simulink model "PAC_experiment"  (R2025a)
settings: Solver=VariableStepAuto  StartTime=0.0  StopTime=200  RelTol=1e-3
undefined symbols (not defined in the file or in its folder): National_Instruments, PCI
libraries: sldrtlib x3, simulink x1
settings Model: Creator=dperera  LastModifiedBy=dperera

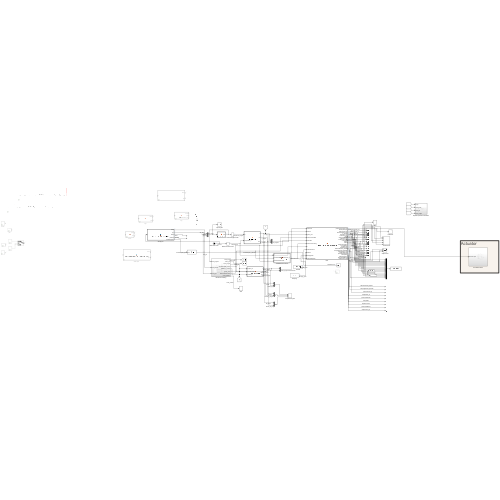
[thumbnail: Simulink's stored preview of the top-level diagram]
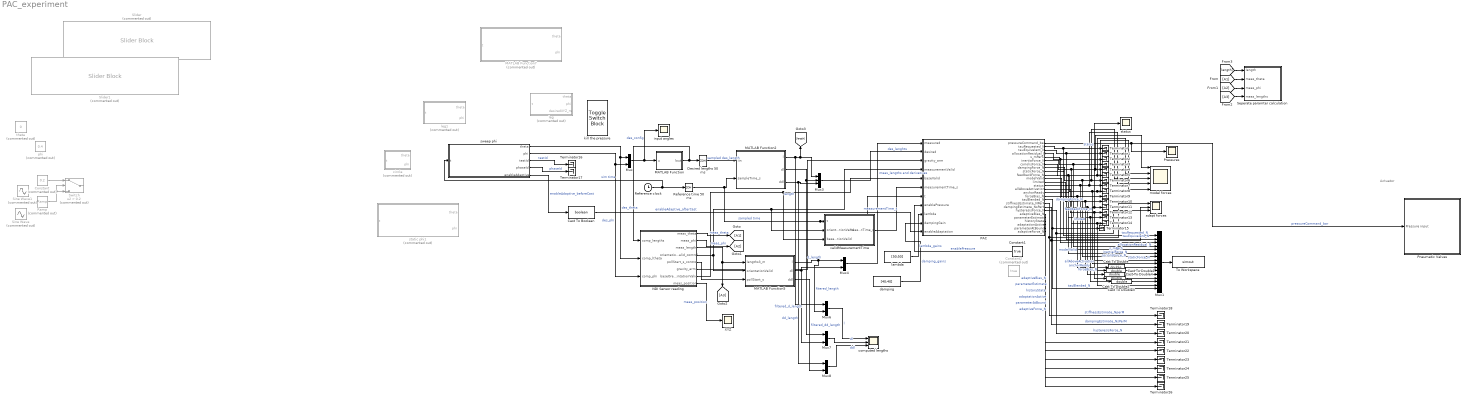
== system PAC_experiment ==
  note: Actuator
  Cast To Boolean : DataTypeConversion  OutDataTypeStr=boolean  SaturateOnIntegerOverflow=off  RndMeth=Floor
  Cast To Double{,1..4} (5 alike) : DataTypeConversion  OutDataTypeStr=double  SaturateOnIntegerOverflow=off  RndMeth=Floor
  Constant : Constant  Commented=on  Value=0.2
  Constant1 : Constant  Value=true  OutDataTypeStr=boolean  SampleTime=0.05
  Constant2 : Constant  Commented=on  Value=true  OutDataTypeStr=boolean
  Desired lengths 50 ms : ZeroOrderHold  SampleTime=0.05
  MATLAB Function : MATLAB Function  TreatAsAtomicUnit=on
  MATLAB Function2 : MATLAB Function  TreatAsAtomicUnit=on
  MATLAB Function5 : MATLAB Function  TreatAsAtomicUnit=on
  MATLAB Function7 : MATLAB Function  Commented=on  TreatAsAtomicUnit=on
  Mux{,4,6..8} (5 alike) : Mux  Inputs=2
  Mux1 : Mux  Inputs=16
  Mux3 : Mux  Inputs=3
  NDI Sensor reading : Subsystem
  PAC : MATLAB Function  TreatAsAtomicUnit=on
  Pneumatic Valves : Subsystem
  Pressures : Scope
      settings: ActiveDisplayYMinimum=-0.31343140031485434  ActiveDisplayYMaximum=2.8208826028336897  DataLoggingVariableName=ScopeData6
  Ramp : simulink/Sources/Ramp  Commented=on  slope=0.2/5  start=1  InitialOutput=0
  Reference clock : Clock
  Reference time 50 ms : ZeroOrderHold  SampleTime=0.05
  Seperate paramter calculation : Subsystem
  Sine Wave : Sin  Commented=on  Amplitude=1.5  Bias=1.5  Frequency=0.2  Phase=3*pi/2  SampleTime=0
  Sine Wave1 : Sin  Commented=on  Amplitude=1.5  Bias=1.5  Frequency=0.2  Phase=3*pi/2  SampleTime=0
  Slider : SliderBlock  Commented=on  ScaleMin=-3.14  ScaleMax=3.14
  Slider1 : SliderBlock  Commented=on  ScaleMax=3.14
  Switch : Switch  Commented=on  Criteria=u2 > Threshold  Threshold=0.2  SaturateOnIntegerOverflow=off  InputSameDT=off
  Terminator{,1..26} (27 alike) : Terminator
  To Workspace : ToWorkspace  VariableName=simout  SaveFormat=Timeseries  SampleTime=-1
  XYZ : Scope
      settings: ActiveDisplayYMinimum=-0.091510816574096682  ActiveDisplayYMaximum=0.32359734916687011  DataLoggingVariableName=ScopeData15
  adapt forces : Scope  NumInputPorts=3
      settings: ActiveDisplayYMinimum=-220.00137487802235  ActiveDisplayYMaximum=1980.0123739022017  DataLoggingVariableName=ScopeData9
  circle : MATLAB Function  Commented=on  TreatAsAtomicUnit=on
  computed lengths : Scope  NumInputPorts=3
      settings: ActiveDisplayYMinimum=-0.010198711471822551  ActiveDisplayYMaximum=0.014062901771668192  DataLoggingVariableName=ScopeData11
  damping : Constant  Value=[40;40]  SampleTime=0.05
  input angles : Scope
      settings: ActiveDisplayYMinimum=-0.19634954084936201  ActiveDisplayYMaximum=1.7671458676442586  DataLoggingVariableName=ScopeData12
  kill the pressure : ToggleSwitchBlock
  lambda : Constant  Value=[50;50]  SampleTime=0.05
  leg : MATLAB Function  Commented=on  TreatAsAtomicUnit=on
  leg1 : MATLAB Function  Commented=on  TreatAsAtomicUnit=on
  model forces : Scope  NumInputPorts=5
      settings: ActiveDisplayYMinimum=-0.19318846896969427  ActiveDisplayYMaximum=0.18409547566465151  DataLoggingVariableName=ScopeData10
  phi : Constant  Commented=on  Value=0.4
  static phi1 : MATLAB Function  Commented=on  TreatAsAtomicUnit=on
  status : Scope
      settings: ActiveDisplayYMinimum=-0.49999999999999989  ActiveDisplayYMaximum=4.5  DataLoggingVariableName=ScopeData8
  sweep phi : MATLAB Function  TreatAsAtomicUnit=on
  theta : Constant  Commented=on  Value=0
  validMeasurementTime : MATLAB Function  TreatAsAtomicUnit=on
  wires:
  Mux/1 -> input angles/1, MATLAB Function/1(u)  "des_config"
  MATLAB Function/1(lout) -> Desired lengths 50 ms/1, NDI Sensor reading/1(comp_lengths)
  NDI Sensor reading/3(meas_length) -> MATLAB Function5/1(lengths3_m), [A3]
  MATLAB Function2/1(l) -> Mux6/1, Mux3/1, [length]  "length"
  MATLAB Function2/2(dl) -> Mux7/1, Mux3/2  "d_length"
  MATLAB Function2/3(ddl) -> Mux8/1, Mux3/3  "dd_length"
  MATLAB Function5/1(l) -> Mux6/2, Mux4/1  "fitered_length"
  MATLAB Function5/2(dl) -> Mux7/2, Mux4/2  "filtered_d_length"
  MATLAB Function5/3(ddl) -> Mux8/2  "filtered_dd_length"
  Desired lengths 50 ms/1 -> MATLAB Function2/1(lIn)  "sampled des_length"
  Reference clock/1 -> sweep phi/1(t), Reference time 50 ms/1  "sim time"
  Reference time 50 ms/1 -> PAC/7(t), validMeasurementTime/1(t), MATLAB Function2/2(sampleTime_s)  "sampled time"
  NDI Sensor reading/4(orientationValid_control) -> MATLAB Function5/2(orientationValid), validMeasurementTime/2(orientationValid), PAC/4(measurementValid)
  NDI Sensor reading/5(pollStart_s_control) -> MATLAB Function5/3(pollStart_s)
  NDI Sensor reading/1(meas_theta) -> [A1]  "meas_theta"
  [A1] -> Seperate paramter calculation/2(meas_theta)
  NDI Sensor reading/2(meas_phi) -> [A2]  "meas_phi"
  [A2] -> Seperate paramter calculation/3(meas_phi)
  [A3] -> Seperate paramter calculation/4(meas_lengths)
  [length] -> Seperate paramter calculation/1(length)
  Mux6/1 -> computed lengths/1  "l"
  Mux7/1 -> computed lengths/2  "dl"
  Mux8/1 -> computed lengths/3  "ddl"
  Ramp/1 -> Switch/2, Switch/3
  Constant/1 -> Switch/1
  sweep phi/2(phi) -> NDI Sensor reading/3(comp_phi), Mux/2  "des_phi"
  sweep phi/1(theta) -> NDI Sensor reading/2(comp_ltheta), Mux/1  "des_theta"
  NDI Sensor reading/8(meas_position) -> XYZ/1  "meas_position"
  PAC/1(pressureCommand_bar) -> Pressures/1, Pneumatic Valves/1(Pressure input)  "pressureCommand_bar"
  Mux4/1 -> PAC/1(measured)  "meas_lengths and derivatives"
  Mux3/1 -> PAC/2(desired)  "des_lenghts"
  NDI Sensor reading/6(gravity_arm) -> PAC/3(gravity_arm)
  NDI Sensor reading/7(baseOreintationValid) -> validMeasurementTime/3(baseOrientationValid), PAC/5(baseValid)
  validMeasurementTime/1(measurementTime_s) -> PAC/6(measurementTime_s)  "measurementTime_s"
  Constant1/1 -> PAC/8(enablePressure)  "enablePressure"
  PAC/2(tauRequested_N) -> Terminator/1, Mux1/1  "tauRequested_N"
  PAC/3(tauEquivalent_N) -> Terminator1/1, Mux1/2  "tauEquivalent_N"
  PAC/4(allocationResidual_N) -> Terminator2/1, Mux1/3  "allocationResidual_N"
  PAC/5(s_mPerS) -> Mux1/4, Terminator3/1  "s_mPerS"
  PAC/6(inertiaForce_N) -> model forces/1, Terminator4/1, Mux1/5  "inertialForce_N"
  PAC/7(coriolisForce_N) -> model forces/2, Terminator5/1, Mux1/6  "coriolisForce_N"
  PAC/8(dampingForce_N) -> Mux1/7, model forces/3, Terminator6/1  "dampingForce_N"
  PAC/9(staticForce_N) -> model forces/4, Terminator7/1, Mux1/8  "staticForce_N"
  PAC/10(feedbackForce_N) -> Mux1/9, model forces/5, Terminator8/1  "feedbackForce_N"
  PAC/11(modelValid) -> Terminator9/1, Cast To Double/1  "modelValid"
  PAC/12(limited) -> Terminator10/1, Cast To Double1/1  "limited"
  PAC/13(status) -> status/1, Terminator11/1, Cast To Double4/1  "status"
  PAC/14(allAboveActivation) -> Cast To Double2/1, Terminator12/1  "allAboveActivation"
  PAC/15(anchorReady) -> Terminator13/1, Cast To Double3/1  "anchorReady"
  PAC/16(forceBias_N) -> Mux1/15, Terminator14/1  "forceBias_N"
  PAC/17(tauBlended_N) -> Terminator15/1, Mux1/16  "tauBlended_N"
  Mux1/1 -> To Workspace/1
  Cast To Double/1 -> Mux1/10
  Cast To Double1/1 -> Mux1/11
  Cast To Double2/1 -> Mux1/13
  Cast To Double3/1 -> Mux1/14
  Cast To Double4/1 -> Mux1/12
  lambda/1 -> PAC/9(lambda)  "lambda_gains"
  damping/1 -> PAC/10(dampingGain)  "damping_gains"
  PAC/18(stiffnessEstimate_NPerM) -> adapt forces/1, Terminator18/1  "stiffnessEstimate_NperM"
  PAC/19(dampingEstimate_NsPerM) -> adapt forces/2, Terminator19/1  "dampingEstimate_NsPerM"
  PAC/20(hysteresisForce_N) -> adapt forces/3, Terminator20/1  "hysteresisForce_N"
  PAC/21(adaptiveBias_N) -> Terminator21/1  "adaptiveBias_N"
  PAC/22(parameterEstimate) -> Terminator22/1  "parameterEstimate"
  PAC/23(historyState) -> Terminator23/1  "historyState"
  PAC/24(adaptationActive) -> Terminator24/1  "adaptationActive"
  PAC/25(parameterAtBound) -> Terminator25/1  "parameterAtBound"
  PAC/26(adaptiveForce_N) -> Terminator26/1  "adaptiveForce_N"
  sweep phi/3(testId) -> Terminator16/1  "testId"
  sweep phi/4(phaseId) -> Terminator17/1  "phaseId"
  sweep phi/5(enableAdaptive) -> Cast To Boolean/1  "enableAdaptive_beforeCast"
  Cast To Boolean/1 -> PAC/11(enableAdaptation)  "enableAdaptive_afterCast"

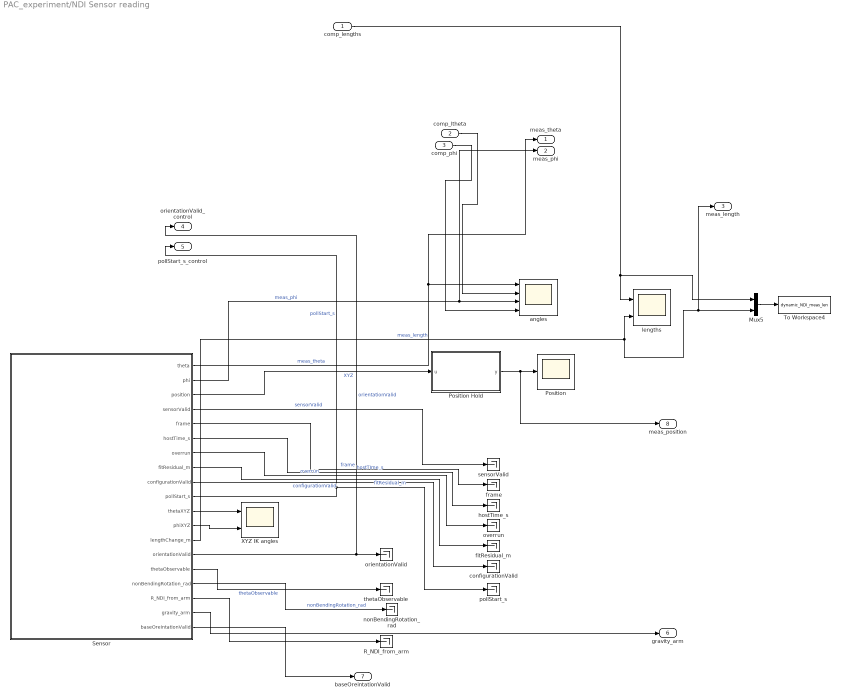
== system PAC_experiment/NDI Sensor reading ==
  comp_lengths : Inport
  comp_ltheta : Inport  Port=2
  comp_phi : Inport  Port=3
  Mux5 : Mux  Inputs=2
  Position : Scope
      settings: ActiveDisplayYMinimum=-0.21656345474719998  ActiveDisplayYMaximum=0.33777835857868188
  Position Hold : MATLAB Function  TreatAsAtomicUnit=on
  R_NDI_from_arm : Terminator
  Sensor : Subsystem
  To Workspace4 : ToWorkspace  VariableName=dynamic_NDI_meas_len  SaveFormat=Timeseries  SampleTime=-1
  XYZ IK angles : Scope  NumInputPorts=2
      settings: DataLoggingVariableName=ScopeData2
  angles : Scope  NumInputPorts=4
      settings: ActiveDisplayYMinimum=-1.199121055664828  ActiveDisplayYMaximum=1.8446149853511815
  configurationValid : Terminator
  fitResidual_m : Terminator
  frame : Terminator
  hostTime_s : Terminator
  lengths : Scope  NumInputPorts=2
      settings: ActiveDisplayYMinimum=-0.0017146774565175815  ActiveDisplayYMaximum=0.0020057370608089205  DataLoggingVariableName=ScopeData3
  nonBendingRotation_rad : Terminator
  orientationValid : Terminator
  overrun : Terminator
  pollStart_s : Terminator
  sensorValid : Terminator
  thetaObservable : Terminator
  meas_theta : Outport
  meas_phi : Outport  Port=2
  meas_length : Outport  Port=3
  orientationValid_control : Outport  Port=4
  pollStart_s_control : Outport  Port=5
  gravity_arm : Outport  Port=6
  baseOreintationValid : Outport  Port=7
  meas_position : Outport  Port=8
  wires:
  Sensor/13(lengthChange_m) -> lengths/2, meas_length/1, Mux5/2  "meas_length"
  comp_lengths/1 -> lengths/1, Mux5/1
  Sensor/10(pollStart_s) -> pollStart_s_control/1, pollStart_s/1  "pollStart_s"
  Sensor/2(phi) -> angles/3, meas_phi/1  "meas_phi"
  Sensor/3(position) -> Position Hold/1(u)  "XYZ"
  Sensor/1(theta) -> meas_theta/1, angles/1  "meas_theta"
  Sensor/6(hostTime_s) -> hostTime_s/1  "hostTIme_s"
  Sensor/9(configurationValid) -> configurationValid/1  "configurationValid"
  Sensor/4(sensorValid) -> sensorValid/1  "sensorValid"
  Sensor/7(overrun) -> overrun/1  "overrun"
  Sensor/5(frame) -> frame/1  "frame"
  comp_ltheta/1 -> angles/2
  Sensor/8(fitResidual_m) -> fitResidual_m/1  "fitResidual_m"
  Sensor/12(phiXYZ) -> XYZ IK angles/2
  Sensor/11(thetaXYZ) -> XYZ IK angles/1
  Position Hold/1(y) -> meas_position/1, Position/1
  Mux5/1 -> To Workspace4/1
  Sensor/14(orientationValid) -> orientationValid_control/1, orientationValid/1  "orientationValid"
  Sensor/16(nonBendingRotation_rad) -> nonBendingRotation_rad/1  "nonBendingRotation_rad"
  Sensor/15(thetaObservable) -> thetaObservable/1  "thetaObservable"
  comp_phi/1 -> angles/4
  Sensor/19(baseOreintationValid) -> baseOreintationValid/1
  Sensor/17(R_NDI_from_arm) -> R_NDI_from_arm/1
  Sensor/18(gravity_arm) -> gravity_arm/1

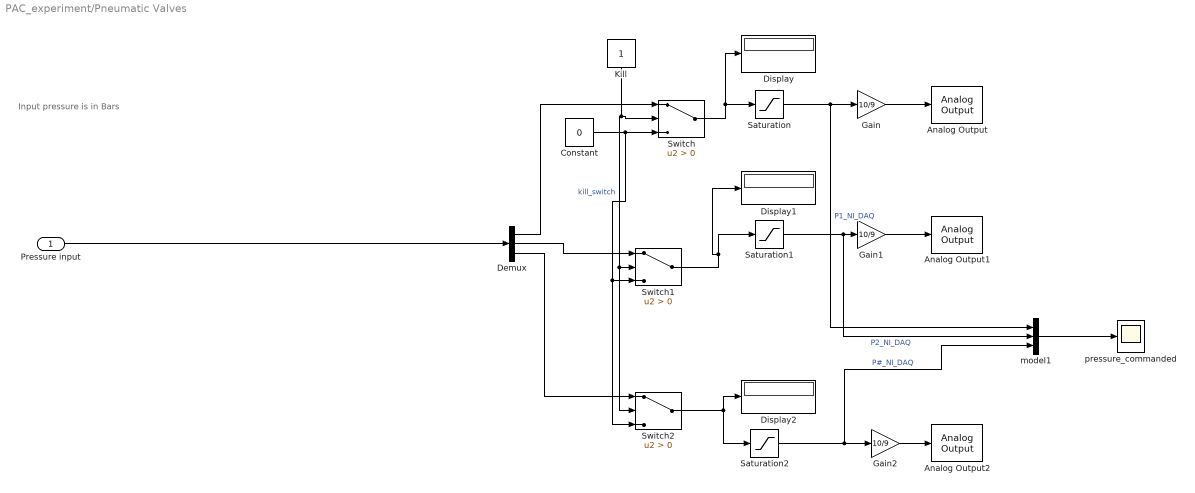
== system PAC_experiment/Pneumatic Valves ==
  note: Input pressure is in Bars
  Pressure input : Inport
  Analog Output : sldrtlib/Analog Output  SampleTime=1/100  MaxMissedTicks=inf  ShowMissedTicks=off  YieldWhenWaiting=off  DrvName=National_Instruments/PCI-6703  DrvAddress=4294967295  DrvOptions=0  Channels=1  RangeMode=1  VoltRange=1  InitialValue=0  FinalValue=0
      settings: AttributesFormatString=National Instruments\nPCI-6703 [auto]
  Analog Output1 : sldrtlib/Analog Output  SampleTime=1/100  MaxMissedTicks=inf  ShowMissedTicks=off  YieldWhenWaiting=off  DrvName=National_Instruments/PCI-6703  DrvAddress=4294967295  DrvOptions=0  Channels=2  RangeMode=1  VoltRange=1  InitialValue=0  FinalValue=0
      settings: AttributesFormatString=National Instruments\nPCI-6703 [auto]
  Analog Output2 : sldrtlib/Analog Output  SampleTime=1/100  MaxMissedTicks=inf  ShowMissedTicks=off  YieldWhenWaiting=off  DrvName=National_Instruments/PCI-6703  DrvAddress=4294967295  DrvOptions=0  Channels=3  RangeMode=1  VoltRange=1  InitialValue=0  FinalValue=0
      settings: AttributesFormatString=National Instruments\nPCI-6703 [auto]
  Constant : Constant  Value=0
  Demux : Demux  Outputs=3
  Display : Display
  Display1 : Display
  Display2 : Display
  Gain : Gain  Gain=10/9
  Gain1 : Gain  Gain=10/9
  Gain2 : Gain  Gain=10/9
  Kill : Constant
  Saturation : Saturate  UpperLimit=3  LowerLimit=0
  Saturation1 : Saturate  UpperLimit=3  LowerLimit=0
  Saturation2 : Saturate  UpperLimit=3  LowerLimit=0
  Switch : Switch  Criteria=u2 > Threshold  SaturateOnIntegerOverflow=off  InputSameDT=off
  Switch1 : Switch  Criteria=u2 > Threshold  SaturateOnIntegerOverflow=off  InputSameDT=off
  Switch2 : Switch  Criteria=u2 > Threshold  SaturateOnIntegerOverflow=off  InputSameDT=off
  model1 : Mux  Inputs=3
  pressure_commanded : Scope
      settings: ActiveDisplayYMinimum=-0.37499999999999989  ActiveDisplayYMaximum=3.375  DataLoggingVariableName=ScopeData7
  wires:
  Constant/1 -> Switch2/3, Switch1/3, Switch/3
  Kill/1 -> Switch2/2, Switch1/2, Switch/2  "kill_switch"
  Switch/1 -> Display/1, Saturation/1
  Gain/1 -> Analog Output/1
  Saturation/1 -> model1/1, Gain/1  "P1_NI_DAQ"
  Demux/3 -> Switch2/1
  Gain1/1 -> Analog Output1/1
  Gain2/1 -> Analog Output2/1
  Saturation2/1 -> model1/3, Gain2/1  "P#_NI_DAQ"
  Switch2/1 -> Saturation2/1, Display2/1
  Demux/2 -> Switch1/1
  Switch1/1 -> Saturation1/1, Display1/1
  model1/1 -> pressure_commanded/1
  Saturation1/1 -> model1/2, Gain1/1  "P2_NI_DAQ"
  Demux/1 -> Switch/1
  Pressure input/1 -> Demux/1

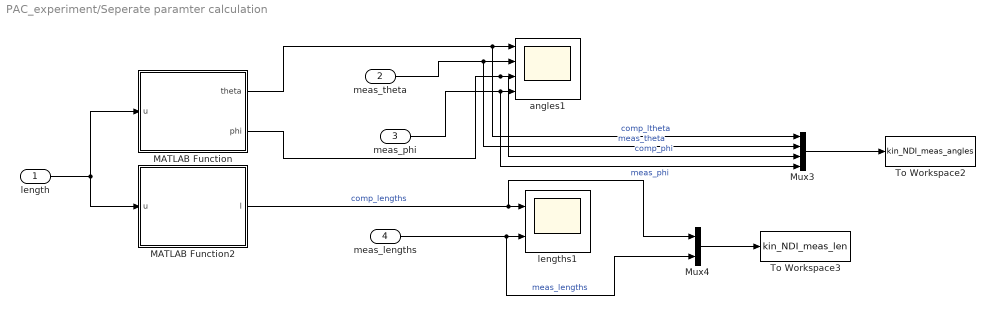
== system PAC_experiment/Seperate paramter calculation ==
  length : Inport
  meas_theta : Inport  Port=2
  meas_phi : Inport  Port=3
  meas_lengths : Inport  Port=4
  MATLAB Function : MATLAB Function  TreatAsAtomicUnit=on
  MATLAB Function2 : MATLAB Function  TreatAsAtomicUnit=on
  Mux3 : Mux
  Mux4 : Mux  Inputs=2
  To Workspace2 : ToWorkspace  VariableName=kin_NDI_meas_angles  SaveFormat=Timeseries  SampleTime=-1
  To Workspace3 : ToWorkspace  VariableName=kin_NDI_meas_len  SaveFormat=Timeseries  SampleTime=-1
  angles1 : Scope  NumInputPorts=4
      settings: ActiveDisplayYMinimum=-3.9269137322662839  ActiveDisplayYMaximum=3.9265599408279468  DataLoggingVariableName=ScopeData4
  lengths1 : Scope  NumInputPorts=2
      settings: ActiveDisplayYMinimum=-0.02243223759551808  ActiveDisplayYMaximum=0.037530111947788623  DataLoggingVariableName=ScopeData5
  wires:
  meas_lengths/1 -> Mux4/2, lengths1/2  "meas_lengths"
  meas_theta/1 -> Mux3/2, angles1/2  "meas_theta"
  MATLAB Function/2(phi) -> Mux3/3, angles1/3  "comp_phi"
  Mux3/1 -> To Workspace2/1
  meas_phi/1 -> Mux3/4, angles1/4  "meas_phi"
  MATLAB Function/1(theta) -> Mux3/1, angles1/1  "comp_ltheta"
  Mux4/1 -> To Workspace3/1
  MATLAB Function2/1(l) -> Mux4/1, lengths1/1  "comp_lengths"
  length/1 -> MATLAB Function2/1(u), MATLAB Function/1(u)

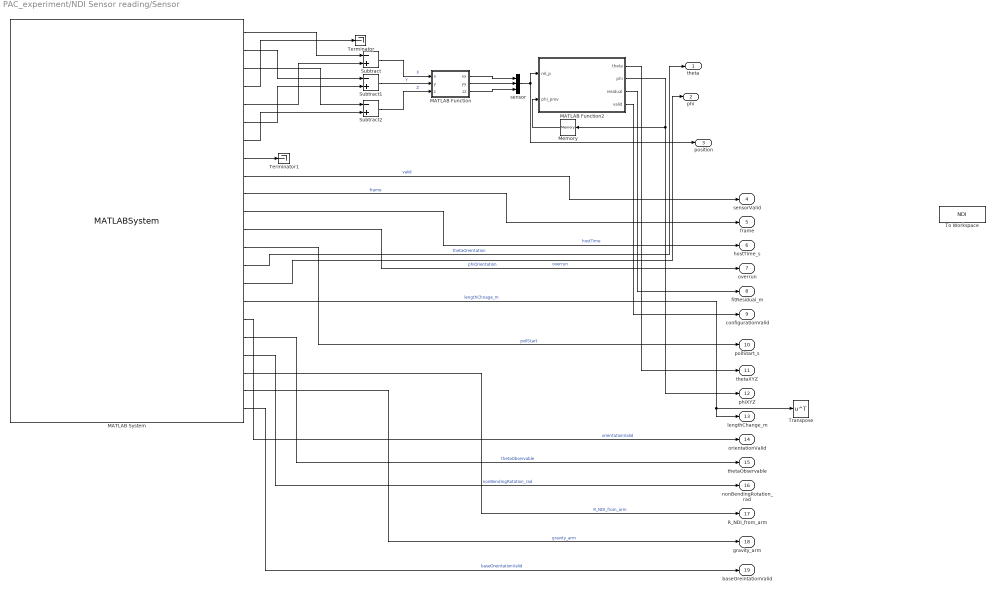
== system PAC_experiment/NDI Sensor reading/Sensor ==
  MATLAB Function : MATLAB Function  TreatAsAtomicUnit=on
  MATLAB Function2 : MATLAB Function  TreatAsAtomicUnit=on
  MATLAB System : MATLABSystem  System=AuroraReader_s2_BaseRotation  Port=COM12  BaudRate=921600  SamplePeriod=0.05  BaseSensorId=0A  TipSensorId=0B  CalibrationFile=C:\Users\dperera\OneDrive - Texas A&M University\Lab\Research\fDyn_ExpCom\hyDyn_Ctrl\ndi_orientation_recordings\calibration_20260930_190505_898.mat  PreflightSeconds=5  ActuatorRadius=0.013  ReferenceGravity_arm=[ 0; 0; -9.81 ]  SimulateUsing=Interpreted execution
      mask Type: AuroraReader_s2_BaseRotation
  Memory : Memory  InitialCondition=0.0001
  Subtract : Sum  Inputs=-+
  Subtract1 : Sum  Inputs=-+
  Subtract2 : Sum  Inputs=-+
  Terminator : Terminator
  Terminator1 : Terminator
  To Workspace : ToWorkspace  VariableName=NDI  SaveFormat=Timeseries  SampleTime=-1
  Transpose : Math  Operator=transpose
  sensor : Mux  Inputs=3
  theta : Outport
  phi : Outport  Port=2
  position : Outport  Port=3
  sensorValid : Outport  Port=4
  frame : Outport  Port=5
  hostTime_s : Outport  Port=6
  overrun : Outport  Port=7
  fitResidual_m : Outport  Port=8
  configurationValid : Outport  Port=9
  pollStart_s : Outport  Port=10
  thetaXYZ : Outport  Port=11
  phiXYZ : Outport  Port=12
  lengthChange_m : Outport  Port=13
  orientationValid : Outport  Port=14
  thetaObservable : Outport  Port=15
  nonBendingRotation_rad : Outport  Port=16
  R_NDI_from_arm : Outport  Port=17
  gravity_arm : Outport  Port=18
  baseOreintationValid : Outport  Port=19
  wires:
  MATLAB System/2 -> Subtract1/1
  MATLAB Function/3(zz) -> sensor/3
  Subtract1/1 -> MATLAB Function/2(y)  "Y"
  Subtract2/1 -> MATLAB Function/3(z)  "Z"
  MATLAB System/5 -> Subtract/2
  sensor/1 -> position/1, MATLAB Function2/1(rel_p)
  MATLAB System/8 -> Terminator1/1
  MATLAB Function/1(xx) -> sensor/1
  Subtract/1 -> MATLAB Function/1(x)  "X"
  MATLAB Function/2(yy) -> sensor/2
  MATLAB System/1 -> Subtract/1
  MATLAB Function2/2(phi) -> Memory/1, phiXYZ/1
  MATLAB System/7 -> Subtract2/2
  MATLAB System/4 -> Terminator/1
  MATLAB System/3 -> Subtract2/1
  MATLAB System/6 -> Subtract1/2
  Memory/1 -> MATLAB Function2/2(phi_prev)
  MATLAB System/9 -> sensorValid/1  "valid"
  MATLAB System/11 -> hostTime_s/1  "hostTime"
  MATLAB System/12 -> overrun/1  "overrun"
  MATLAB Function2/3(residual) -> fitResidual_m/1
  MATLAB Function2/4(valid) -> configurationValid/1
  MATLAB System/13 -> pollStart_s/1  "pollStart"
  MATLAB System/14 -> theta/1  "thetaOrientation"
  MATLAB System/15 -> phi/1  "phiOrientation"
  MATLAB Function2/1(theta) -> thetaXYZ/1
  MATLAB System/16 -> lengthChange_m/1, Transpose/1  "lengthChnage_m"
  MATLAB System/17 -> orientationValid/1  "orientationValid"
  MATLAB System/18 -> thetaObservable/1  "thetaObservable"
  MATLAB System/19 -> nonBendingRotation_rad/1  "nonBendingRotation_rad"
  MATLAB System/10 -> frame/1  "frame"
  MATLAB System/20 -> R_NDI_from_arm/1  "R_NDI_from_arm"
  MATLAB System/21 -> gravity_arm/1  "gravity_arm"
  MATLAB System/22 -> baseOreintationValid/1  "baseOreintationValid"

== matlab function PAC_experiment/Seperate paramter calculation/MATLAB Function ==
  data: u input; theta output; phi output
function [theta, phi] = length2config(u)
%#codegen
% This file convert the length changes into theta/phi
%
% Inputs:
%   u       : length change[2x1] (m)
%             [l2; l3]
%
% Outputs:
%   theta   : bending direction [constant] (rad)
%   phi     : bending amount [constant] (rad)

l = [0.0; u(1); u(2)];
r  = 0.013;

c = [atan2(l(3) - l(2), sqrt(0.3e1) * (l(2) + l(3)));
    0.2e1 / 0.3e1 / r * sqrt((3 * l(2) ^ 2 + 3 * l(3) * l(2) + 3 * l(3) ^ 2))];

theta = c(1);
phi = c(2);

end

== matlab function PAC_experiment/Seperate paramter calculation/MATLAB Function2 ==
  data: u input; l output
function l = lengthVector(u)
%#codegen
% This file create the length vector
%
% Inputs:
%   u       : length change[2x1] (m)
%             [l2; l3]
%
% Outputs:
%   l   : bending direction [3x1] (m)

l = [-(u(1) + u(2)); u(1); u(2)];

end

== matlab function PAC_experiment/NDI Sensor reading/Position Hold ==
  data: u input; y output
function y = fcn(u)
persistent lastPosition
if isempty(lastPosition), lastPosition=nan(3,1); end
if all(isfinite(u)), lastPosition=u; end
y=lastPosition;
end

== matlab function PAC_experiment/NDI Sensor reading/Sensor/MATLAB Function ==
  data: x input; xx output; y input; z input; yy output; zz output
function [xx,yy,zz] = rotateX90(x,y,z)

    R = [1 0 0;
         0 0 1;
         0 -1 0];

    p = R*[x;y;z]*0.001;

    xx=p(1);
    yy=p(2);
    zz=p(3);

    
end

== matlab function PAC_experiment/NDI Sensor reading/Sensor/MATLAB Function2 ==
  data: rel_p input; theta output; phi output; phi_prev input; residual output; valid output
function [theta,phi,residual,valid] = xyz2ThetaPhi(rel_p,phi_prev)
persistent lastPhi lastTheta lastOutputTheta lastOutputPhi lastResidual
if isempty(lastPhi)
    lastPhi=0.0001; lastTheta=0;
    lastOutputTheta=NaN; lastOutputPhi=NaN; lastResidual=NaN;
end
% Keep the external memory for compatibility; never use its NaN.
if isfinite(phi_prev), lastPhi=phi_prev; end
[theta,phi,residual,valid]=ndiSupportFnc.configuration(rel_p,lastPhi,lastTheta);
if valid
    lastPhi=phi; lastTheta=theta;
    lastOutputTheta=theta; lastOutputPhi=phi; lastResidual=residual;
else
    % Scope outputs hold, but configurationValid remains false.
    theta=lastOutputTheta; phi=lastOutputPhi; residual=lastResidual;
end
end

== matlab function PAC_experiment/MATLAB Function ==
  data: u input; lout output
function lout = config2length(u)
%#codegen
% Convert configuration variables to length changes
% Input (u):
%   u       : theta and phi [2x1] (rad)
%               theta angle (rad) [constant]
%               phi angle (rad) [constant]
%   r       : radial offset (m) [constant]
% 
% Output:
%   lout    : lenght changes (m) [s,1]


theta = u(1);
phi = u(2);
r = 0.013;

l = [-r * cos(theta) * phi;
    (0.5e0 * r * cos(theta) - sqrt(0.3e1) * r * sin(theta) / 0.2e1) * phi;
    (0.5e0 * r * cos(theta) + sqrt(0.3e1) * r * sin(theta) / 0.2e1) * phi];

lout = [l(2); l(3)];

end

== matlab function PAC_experiment/MATLAB Function2 ==
  data: lIn input; l output; dl output; ddl output; sampleTime_s input
function [l, dl, ddl] = lengthDerivatives(lIn, sampleTime_s)
%#codegen
% Desired reduced lengths [l2;l3] in m; derivatives in m/s and m/s^2.
% sampleTime_s is a 0.05 s zero-order-held Clock signal.
persistent lastL lastT velocity acceleration
if isempty(lastT)
    lastL = zeros(2,1);
    lastT = -1;
    velocity = zeros(2,1);
    acceleration = zeros(2,1);
end
l = lastL;
dl = velocity;
ddl = acceleration;
if ~all(isfinite(lIn)) || ~isfinite(sampleTime_s)
    return;
end
q = [lIn(1); lIn(2)];
if lastT < 0
    lastL = q;
    lastT = sampleTime_s;
    l = q;
    return;
end
dt = sampleTime_s - lastT;
if dt > 1e-6
    rawVelocity = (q-lastL)/dt;
    oldVelocity = velocity;
    alphaV = dt/(0.10+dt);
    velocity = velocity + alphaV*(rawVelocity-velocity);
    rawAcceleration = (velocity-oldVelocity)/dt;
    alphaA = dt/(0.15+dt);
    acceleration = acceleration + alphaA*(rawAcceleration-acceleration);
    lastL = q;
    lastT = sampleTime_s;
end
l = lastL;
dl = velocity;
ddl = acceleration;
end

== matlab function PAC_experiment/validMeasurementTime ==
  data: t input; measurementTime_s output; orientationValid input; baseOrientationValid input
function measurementTime_s = validMeasurementTime( ...
    t, orientationValid, baseOrientationValid)
%#codegen

persistent lastValidTime
if isempty(lastValidTime)
    lastValidTime = -1.0;
end

if orientationValid && baseOrientationValid && isfinite(t)
    lastValidTime = t;
end

measurementTime_s = lastValidTime;
end

== matlab function PAC_experiment/sweep phi ==
  data: t input; theta output; phi output; testId output; phaseId output; enableAdaptive output
function [theta,phi,testId,phaseId, enableAdaptive] = pacStaticSweepReferenceBlock(t)
%#codegen
% Paste into reference MATLAB Function block. All settings are internal.
% 10 trials: three amplitudes in three directions, then repeat theta=0/.2.
% Stop Time 535 s. Start only if controller status=3 before 25 s.
% Learn normally, then freeze before the 0.8-rad unloading at 110 s.
adaptationFreezeTime_s = 105.0;
enableAdaptive = isfinite(t) && t >= 0.0 && ...
                 t < adaptationFreezeTime_s;
start_s=25.0;
rise_s=5.0; hold_s=30.0; fall_s=5.0; zeroHold_s=10.0;
thetaList=[0 0 0 pi/2 pi/2 pi/2 pi pi pi 0];
phiList=[.5 .8 1.0 .5 .8 1.0 .5 .8 1.0 .5];
theta=0.0;phi=0.0;testId=0.0;phaseId=0.0;
if ~isfinite(t) || t<start_s, return; end
trial_s=rise_s+hold_s+fall_s+zeroHold_s;
idx=floor((t-start_s)/trial_s)+1;
if idx>numel(phiList),return;end
testId=double(idx);theta=thetaList(idx);
local=t-start_s-(idx-1)*trial_s;
if local<rise_s
    phaseId=1.0;u=local/rise_s;phi=phiList(idx)*u*u*(3-2*u);
elseif local<rise_s+hold_s
    phaseId=2.0;phi=phiList(idx);
elseif local<rise_s+hold_s+fall_s
    phaseId=3.0;u=(local-rise_s-hold_s)/fall_s;
    phi=phiList(idx)*(1-u*u*(3-2*u));
else
    phaseId=4.0;
end
end

== matlab function PAC_experiment/MATLAB Function5 ==
  data: lengths3_m input; l output; dl output; ddl output; orientationValid input; pollStart_s input
function [l, dl, ddl] = filteredDerivatives(lengths3_m, orientationValid, pollStart_s)
%#codegen
% NDI lengths are [l1;l2;l3]; model coordinates are [l2;l3].
% Invalid or repeated BX frames do not update the derivative states.
persistent lastL lastT velocity acceleration
if isempty(lastT)
    lastL = nan(2,1);
    lastT = -1;
    velocity = zeros(2,1);
    acceleration = zeros(2,1);
end
l = lastL;
dl = velocity;
ddl = acceleration;
if ~orientationValid || ~all(isfinite(lengths3_m)) || ~isfinite(pollStart_s)
    return;
end
q = [lengths3_m(2); lengths3_m(3)];
if lastT < 0
    lastL = q;
    lastT = pollStart_s;
    l = q;
    return;
end
dt = pollStart_s-lastT;
if dt > 1e-6
    rawVelocity = (q-lastL)/dt;
    oldVelocity = velocity;
    alphaV = dt/(0.20+dt);
    velocity = velocity + alphaV*(rawVelocity-velocity);
    rawAcceleration = (velocity-oldVelocity)/dt;
    alphaA = dt/(0.30+dt);
    acceleration = acceleration + alphaA*(rawAcceleration-acceleration);
    lastL = q;
    lastT = pollStart_s;
end
l = lastL;
dl = velocity;
ddl = acceleration;
end

== matlab function PAC_experiment/static phi1 ==
  data: t input; theta output; phi output
function [theta, phi] = commonPressureFeedbackReferenceBlock(t)
%#codegen
% Fixed-direction ramp-and-hold test.
% Suggested simulation Stop Time: 70 s.

des_phi = 0.2;       % rad
des_theta = 0.0;     % rad
startTime_s = 25.0;  % Allow trim and feedback blend to finish
riseTime_s = 5.0;
holdTime_s = 30.0;
fallTime_s = 5.0;

theta = des_theta;
phi = 0.0;

if ~isfinite(t) || t < 0.0
    return;
end

holdStart_s = startTime_s + riseTime_s;
fallStart_s = holdStart_s + holdTime_s;
endTime_s = fallStart_s + fallTime_s;

if t < startTime_s
    return;
elseif t < holdStart_s
    u = (t - startTime_s)/riseTime_s;
    phi = des_phi*u*u*(3.0 - 2.0*u);
elseif t < fallStart_s
    phi = des_phi;
elseif t < endTime_s
    u = (t - fallStart_s)/fallTime_s;
    phi = des_phi*(1.0 - u*u*(3.0 - 2.0*u));
end
end

== matlab function PAC_experiment/MATLAB Function7 ==
  data: t input; theta output; phi output
function [theta, phi] = commonPressureFeedbackReferenceBlock(t)
%#codegen
% Paste into the existing thetaCircle MATLAB Function block in a COPY of
% the feedback-linearization model. Connect theta and phi to the desired
% angle Mux and NDI comparison inputs; bypass the old circle/ramp sources.
% Stop Time: 240 s. Both reference steps are only 0.01 rad.

theta = 0.0;
phi = 0.0;
if ~isfinite(t) || t < 0.0
    return;
end

if t >= 90.0 && t < 130.0
    theta = 0.0; % U-direction bend.
    if t < 95.0
        u = (t-90.0)/5.0;
        phi = 0.01*u*u*(3.0-2.0*u);
    elseif t < 125.0
        phi = 0.01;
    else
        u = (t-125.0)/5.0;
        phi = 0.01*(1.0-u*u*(3.0-2.0*u));
    end
elseif t >= 160.0 && t < 200.0
    theta = pi/2; % V-direction bend.
    if t < 165.0
        u = (t-160.0)/5.0;
        phi = 0.01*u*u*(3.0-2.0*u);
    elseif t < 195.0
        phi = 0.01;
    else
        u = (t-195.0)/5.0;
        phi = 0.01*(1.0-u*u*(3.0-2.0*u));
    end
end
end

== matlab function PAC_experiment/leg ==
  data: t input; theta output; phi output; desiredXYZ_m output
function [theta, phi, desiredXYZ_m] = square(t)
%#codegen
% One 10 cm x 10 cm square in arm-frame X-Y.
% Z follows the fixed-length, constant-curvature geometry.

side_m = 0.10;
h = side_m/2;

rotationTime_s = 10.0;
trimTime_s = 5.0;
approachTime_s = 10.0;
cornerHold_s = 5.0;
sideTime_s = 5.0;      % time for each 10 cm side
numSquares = 10;         % increase after the first test
returnTime_s = 10.0;

% Base-sensor offset, module length, tip-sensor offset.
Lbase = 0.055;
Lmodule = 0.17411;
Ltip = 0.05;

approachStart_s = rotationTime_s + trimTime_s;
approachEnd_s = approachStart_s + approachTime_s;
squareStart_s = approachEnd_s + cornerHold_s;
squareEnd_s = squareStart_s + 4*numSquares*sideTime_s;
returnEnd_s = squareEnd_s + returnTime_s;

theta = 0.0;
phi = 0.0;
desiredXYZ_m = [0.0; 0.0; Lbase + Lmodule + Ltip];

if ~isfinite(t) || t < approachStart_s
    return;
end

x = 0.0;
y = 0.0;

if t < approachEnd_s
    % Move from straight to the first corner (+h,+h).
    u = (t - approachStart_s)/approachTime_s;
    s = smooth5(u);
    x = h*s;
    y = h*s;
    theta = pi/4;

elseif t < squareStart_s
    % Settle at the first corner.
    x = h;
    y = h;
    theta = pi/4;

elseif t < squareEnd_s
    elapsed = t - squareStart_s;
    lap = floor(elapsed/(4*sideTime_s));
    withinLap = elapsed - lap*(4*sideTime_s);
    side = floor(withinLap/sideTime_s);  % 0, 1, 2, or 3
    u = (withinLap - side*sideTime_s)/sideTime_s;
    s = smooth5(u);

    if side == 0
        x = h - 2*h*s;  y = h;           % (+,+) to (-,+)
    elseif side == 1
        x = -h;         y = h - 2*h*s;   % (-,+) to (-,-)
    elseif side == 2
        x = -h + 2*h*s; y = -h;          % (-,-) to (+,-)
    else
        x = h;          y = -h + 2*h*s;  % (+,-) to (+,+)
    end

    % Keep theta continuous across +/-pi and across laps.
    theta = atan2(y,x);
    if side == 1 && theta < 0.0
        theta = theta + 2*pi;
    elseif side >= 2
        theta = theta + 2*pi;
    end
    theta = theta + 2*pi*lap;

elseif t < returnEnd_s
    % Return from the first corner to straight.
    u = (t - squareEnd_s)/returnTime_s;
    s = smooth5(u);
    x = h*(1.0 - s);
    y = h*(1.0 - s);
    theta = pi/4 + 2*pi*numSquares;

else
    % Remain straight without resetting the unwrapped theta.
    theta = pi/4 + 2*pi*numSquares;
    return;
end

[phi, z] = task2ConfigOnSurface(hypot(x,y), Lbase, Lmodule, Ltip);
desiredXYZ_m = [x; y; z];
end

function s = smooth5(u)
% Zero velocity and acceleration at both ends of each side.
u = min(max(u,0.0),1.0);
s = u*u*u*(10.0 + u*(-15.0 + 6.0*u));
end

function [phi,z] = task2ConfigOnSurface(rho,Lbase,Lmodule,Ltip)
% Invert the same constant-curvature radial geometry as task2config.
% Z is free and is computed from the resulting bend angle.
if rho <= 1e-10
    phi = 0.0;
    z = Lbase + Lmodule + Ltip;
    return;
end

low = 0.0;
high = 1.5;  % rad; comfortably covers this 10 cm square

for k = 1:28
    mid = 0.5*(low + high);
    rhoModel = Lmodule*2.0*sin(mid/2.0)^2/mid ...
             + Ltip*sin(mid);
    if rhoModel < rho
        low = mid;
    else
        high = mid;
    end
end

phi = 0.5*(low + high);
z = Lbase + Lmodule*sin(phi)/phi + Ltip*cos(phi);
end

== matlab function PAC_experiment/circle ==
  data: t input; theta output; phi output
function [theta, phi] = thetaCircle(t)
%#codegen

% Change these values before a run
des_phi = 1.0;             % rad
circle_time_s = 10.0;      % seconds per circle
num_circles = 1;
rotationTime_s = 10.0;     % time available to rotate the base
trimTime_s = 5.0;         % stationary pressure-trim hold
feedbackBlendTime_s = 5.0;
phiRiseTime_s = 5.0;
phiFallTime_s = 5.0;

theta = 0.0;
phi = 0.0;
if ~isfinite(t) || t < 0.0
    return;
end

phiRiseStart_s = rotationTime_s + trimTime_s + feedbackBlendTime_s;
circleStart_s = phiRiseStart_s + phiRiseTime_s;
circleEnd_s = circleStart_s + num_circles*circle_time_s;
phiEnd_s = circleEnd_s + phiFallTime_s;

if t < phiRiseStart_s
    return;
elseif t < circleStart_s
    u = (t - phiRiseStart_s)/phiRiseTime_s;
    phi = des_phi*u*u*(3.0 - 2.0*u);
elseif t < circleEnd_s
    progress = (t - circleStart_s)/circle_time_s;
    lap = floor(progress);
    u = progress - lap;
    theta = 2*pi*(lap + u*u*(3.0 - 2.0*u));
    phi = des_phi;
elseif t < phiEnd_s
    u = (t - circleEnd_s)/phiFallTime_s;
    theta = 2*pi*num_circles;
    phi = des_phi*(1.0 - u*u*(3.0 - 2.0*u));
end
end

== matlab function PAC_experiment/leg1 ==
  data: t input; theta output; phi output
function [theta, phi] = leg(t)
%#codegen

rotationTime_s = 10.0;
trimTime_s = 5.0;
trajectoryStart_s = rotationTime_s + trimTime_s;

% Loaded when the MATLAB Function block compiles.
data = coder.load('Quadruped_leg/Natha_quad_leg_1.mat', ...
                  't', 'leg1_config');
time = data.t;
angles = data.leg1_config;  % row 1: theta; row 2: phi, radians

theta = 0.0;
phi = 0.0;

if ~isfinite(t) || t < trajectoryStart_s
    return;
end

trajectoryTime_s = 0.2 * (t - trajectoryStart_s);

% Hold the final recorded pose after the 40-second trajectory.
if trajectoryTime_s >= time(end)
    theta = angles(1,end);
    phi = angles(2,end);
    return;
end

% Find the two recorded samples surrounding the current time.
lo = 1;
hi = numel(time);
while hi - lo > 1
    mid = floor((lo + hi)/2);
    if trajectoryTime_s < time(mid)
        hi = mid;
    else
        lo = mid;
    end
end

% Linear interpolation between samples.
weight = (trajectoryTime_s - time(lo))/(time(hi) - time(lo));
theta = angles(1,lo) + weight*(angles(1,hi) - angles(1,lo));
phi   = angles(2,lo) + weight*(angles(2,hi) - angles(2,lo));
end

== matlab function PAC_experiment/PAC ==
  settings: sampleTime=0.05
  data: measured input; desired input; gravity_arm input; measurementValid input; baseValid input; measurementTime_s input; t input; pressureCommand_bar output double; tauRequested_N output double; tauEquivalent_N output double; allocationResidual_N output; s_mPerS output; inertiaForce_N output; coriolisForce_N output; dampingForce_N output; staticForce_N output; feedbackForce_N output; modelValid output boolean; limited output boolean; enablePressure input; status output uint8 size=1; allAboveActivation output boolean; anchorReady output boolean; forceBias_N output; tauBlended_N output; lambda input; dampingGain input; enableAdaptation input; stiffnessEstimate_NPerM output; dampingEstimate_NsPerM output; hysteresisForce_N output; adaptiveBias_N output; parameterEstimate output; historyState output; adaptationActive output; parameterAtBound output; adaptiveForce_N output
function [pressureCommand_bar,tauRequested_N,tauEquivalent_N, ...
 allocationResidual_N,s_mPerS,inertiaForce_N,coriolisForce_N, ...
 dampingForce_N,staticForce_N,feedbackForce_N,modelValid,limited, ...
 status,allAboveActivation,anchorReady,forceBias_N,tauBlended_N, ...
 stiffnessEstimate_NPerM,dampingEstimate_NsPerM,hysteresisForce_N, ...
 adaptiveBias_N,parameterEstimate,historyState,adaptationActive, ...
 parameterAtBound,adaptiveForce_N] = pacAdaptiveCommonPressureBlock( ...
 measured,desired,gravity_arm,measurementValid,baseValid,measurementTime_s, ...
 t,enablePressure,lambda,dampingGain,enableAdaptation)
%#codegen
% Paste into NEW controller block; Discrete .05 s. Existing first 8 inputs
% and first 17 outputs preserved. New inputs: lambda 2x1, Ks 2x1, adapt boolean.
% Estimates correspond to force evaluation; updates take effect NEXT sample.
persistent ps as
if isempty(ps),ps=pacPressureInitialState();as=pacAdaptiveInitialState();end
cfg=pacAdaptiveConfig();pc=pacPressureConfig();
good=measurementValid && baseValid && isfinite(measurementTime_s) && ...
 isfinite(t) && measurementTime_s<=t+1e-9 && ...
 t-measurementTime_s<=pc.maxSampleAge_s+1e-9;
dt=0;
if good && measurementTime_s>as.lastSample
 if as.lastSample>=0,dt=measurementTime_s-as.lastSample;end
 if all(isfinite(measured(:))) && ~ps.fault
  as.z=pacAdaptiveHistory(as.z,measured(3:4),dt);
 end
 as.lastSample=measurementTime_s;
end
[tauRequested_N,s_mPerS,Y,inertiaForce_N,coriolisForce_N, ...
 dampingForce_N,staticForce_N,feedbackForce_N,hysteresisForce_N, ...
 adaptiveBias_N,stiffnessEstimate_NPerM,dampingEstimate_NsPerM,modelValid]= ...
 pacAdaptiveForce(measured,desired,gravity_arm,lambda,dampingGain,as,good);
% Capture nominal static+history+bias consistently with current model at trim.
[pressureCommand_bar,tauEquivalent_N,allocationResidual_N,limited,status, ...
 allAboveActivation,tauBlended_N,ps]=pacPressureStep(tauRequested_N, ...
 staticForce_N+hysteresisForce_N+adaptiveBias_N,measured(3:4),modelValid, ...
 measurementTime_s,t,enablePressure,pc,ps);
anchorReady=ps.anchorReady;forceBias_N=ps.forceBias;
parameterEstimate=as.theta;historyState=as.z;
[p,~,~]=pacNominalParameters(gravity_arm);
q=measured(1:2);v=desired(3:4)-lambda(:).*(q-desired(1:2));
adaptiveForce_N=(stiffnessEstimate_NPerM-p.K)*q+ ...
 (dampingEstimate_NsPerM-p.D)*v+hysteresisForce_N+adaptiveBias_N;
allow=enableAdaptation && good && modelValid && status==uint8(3) && ...
 ~limited && all(isfinite(allocationResidual_N)) && ...
 norm(allocationResidual_N)<=cfg.residualTolerance_N;
[as,adaptationActive,parameterAtBound]=pacAdaptiveUpdate(as,Y,s_mPerS,dt,allow);
end
